simulink model "orig_exp3_series"  (R2023a)
settings: Solver=ode4  StartTime=0.0  StopTime=8  FixedStep=0.001  RelTol=1e-3
settings Model: Creator=Anonymous  LastModifiedBy=Anonymous

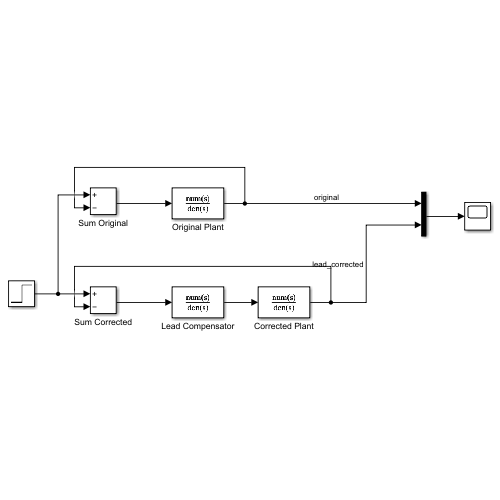
[thumbnail: Simulink's stored preview of the top-level diagram]
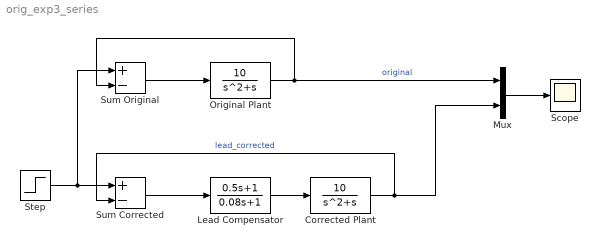
== system orig_exp3_series ==
  Corrected Plant : TransferFcn  Numerator=10  Denominator=[1 1 0]
  Lead Compensator : TransferFcn  Numerator=[0.5 1]  Denominator=[0.08 1]
  Mux : Mux  Inputs=2
  Original Plant : TransferFcn  Numerator=10  Denominator=[1 1 0]
  Scope : Scope
  Step : Step  Time=0  SampleTime=0
  Sum Corrected : Sum  Inputs=+-
  Sum Original : Sum  Inputs=+-
  wires:
  Mux/1 -> Scope/1
  Corrected Plant/1 -> Mux/2, Sum Corrected/2  "lead_corrected"
  Lead Compensator/1 -> Corrected Plant/1
  Sum Corrected/1 -> Lead Compensator/1
  Original Plant/1 -> Mux/1, Sum Original/2  "original"
  Sum Original/1 -> Original Plant/1
  Step/1 -> Sum Corrected/1, Sum Original/1
